simulink model "EV_BMS_SOC"  (R2024a)
settings: Solver=ode1  StartTime=0.0  StopTime=Tstop  FixedStep=Ts  RelTol=1e-3
InitFcn:
  | bms_simulink_init;
values from neighbouring files (symbols this model uses):
  I_max = P_.I_max    [bms_simulink_init.m]
  I_offset = P_.I_offset    [bms_simulink_init.m]
  inv_Cth = 1 / P_.Cth    [bms_simulink_init.m]
  inv_Rth = 1 / P_.Rth    [bms_simulink_init.m]
  k_soc = -100 / (3600 * Q_Ah)    [bms_simulink_init.m]
  OCV_pack = P.OCV_pack    [battery_voltage_model.m]    (also in bms_simulink_init.m = P_.OCV_pack)
  protection_enable = double(sc_.protection)    [bms_simulink_init.m]
  R0 = P_.R0    [bms_simulink_init.m]
  SOC_bp = P.SOC_bp    [battery_voltage_model.m]    (also in bms_simulink_init.m = P_.SOC_bp)
  SOC_init = sc_.SOC_init    [bms_simulink_init.m]
  T_init = sc_.T_init    [bms_simulink_init.m]
  T_max = P_.T_max    [bms_simulink_init.m]
  Ts = P_.dt    [bms_simulink_init.m]
  V_max = P_.V_max    [bms_simulink_init.m]
  V_min = P_.V_min    [bms_simulink_init.m]
undefined symbols (not defined in the file or in its folder): SOC_est_init, stage_select
settings Model: Creator=hp  LastModifiedBy=hp

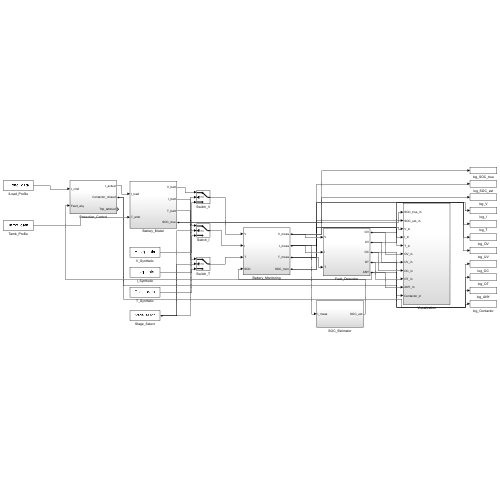
[thumbnail: Simulink's stored preview of the top-level diagram]
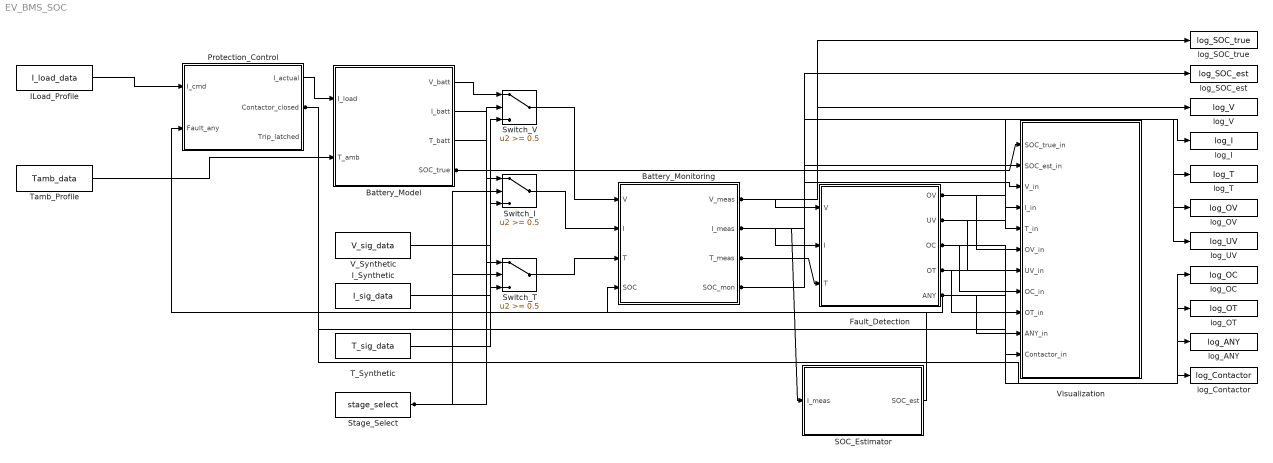
== system EV_BMS_SOC ==
  Battery_Model : Subsystem
  Battery_Monitoring : Subsystem
  Fault_Detection : Subsystem
  ILoad_Profile : FromWorkspace  VariableName=I_load_data  OutputAfterFinalValue=Holding final value
  I_Synthetic : FromWorkspace  VariableName=I_sig_data  OutputAfterFinalValue=Holding final value
  Protection_Control : Subsystem
  SOC_Estimator : Subsystem
  Stage_Select : Constant  Value=stage_select
  Switch_I : Switch  Threshold=0.5  SaturateOnIntegerOverflow=off  InputSameDT=off
  Switch_T : Switch  Threshold=0.5  SaturateOnIntegerOverflow=off  InputSameDT=off
  Switch_V : Switch  Threshold=0.5  SaturateOnIntegerOverflow=off  InputSameDT=off
  T_Synthetic : FromWorkspace  VariableName=T_sig_data  OutputAfterFinalValue=Holding final value
  Tamb_Profile : FromWorkspace  VariableName=Tamb_data  OutputAfterFinalValue=Holding final value
  V_Synthetic : FromWorkspace  VariableName=V_sig_data  OutputAfterFinalValue=Holding final value
  Visualization : Subsystem
  log_ANY : ToWorkspace  VariableName=log_ANY  SampleTime=-1
  log_Contactor : ToWorkspace  VariableName=log_Contactor  SampleTime=-1
  log_I : ToWorkspace  VariableName=log_I  SampleTime=-1
  log_OC : ToWorkspace  VariableName=log_OC  SampleTime=-1
  log_OT : ToWorkspace  VariableName=log_OT  SampleTime=-1
  log_OV : ToWorkspace  VariableName=log_OV  SampleTime=-1
  log_SOC_est : ToWorkspace  VariableName=log_SOC_est  SampleTime=-1
  log_SOC_true : ToWorkspace  VariableName=log_SOC_true  SampleTime=-1
  log_T : ToWorkspace  VariableName=log_T  SampleTime=-1
  log_UV : ToWorkspace  VariableName=log_UV  SampleTime=-1
  log_V : ToWorkspace  VariableName=log_V  SampleTime=-1
  wires:
  ILoad_Profile/1 -> Protection_Control/1(I_cmd)
  Protection_Control/1(I_actual) -> Battery_Model/1(I_load)
  Tamb_Profile/1 -> Battery_Model/2(T_amb)
  Battery_Model/1(V_batt) -> Switch_V/1
  V_Synthetic/1 -> Switch_V/3
  Stage_Select/1 -> Switch_V/2, Switch_I/2, Switch_T/2
  Battery_Model/2(I_batt) -> Switch_I/1
  I_Synthetic/1 -> Switch_I/3
  Battery_Model/3(T_batt) -> Switch_T/1
  T_Synthetic/1 -> Switch_T/3
  Switch_V/1 -> Battery_Monitoring/1(V)
  Switch_I/1 -> Battery_Monitoring/2(I)
  Switch_T/1 -> Battery_Monitoring/3(T)
  SOC_Estimator/1(SOC_est) -> Battery_Monitoring/4(SOC)
  Battery_Monitoring/2(I_meas) -> SOC_Estimator/1(I_meas), Fault_Detection/2(I), Visualization/4(I_in), log_I/1
  Battery_Monitoring/1(V_meas) -> Fault_Detection/1(V), Visualization/3(V_in), log_V/1
  Battery_Monitoring/3(T_meas) -> Fault_Detection/3(T), Visualization/5(T_in), log_T/1
  Fault_Detection/5(ANY) -> Protection_Control/2(Fault_any), Visualization/10(ANY_in), log_ANY/1
  Battery_Model/4(SOC_true) -> Visualization/1(SOC_true_in), log_SOC_true/1
  Battery_Monitoring/4(SOC_mon) -> Visualization/2(SOC_est_in), log_SOC_est/1
  Fault_Detection/1(OV) -> Visualization/6(OV_in), log_OV/1
  Fault_Detection/2(UV) -> Visualization/7(UV_in), log_UV/1
  Fault_Detection/3(OC) -> Visualization/8(OC_in), log_OC/1
  Fault_Detection/4(OT) -> Visualization/9(OT_in), log_OT/1
  Protection_Control/2(Contactor_closed) -> Visualization/11(Contactor_in), log_Contactor/1

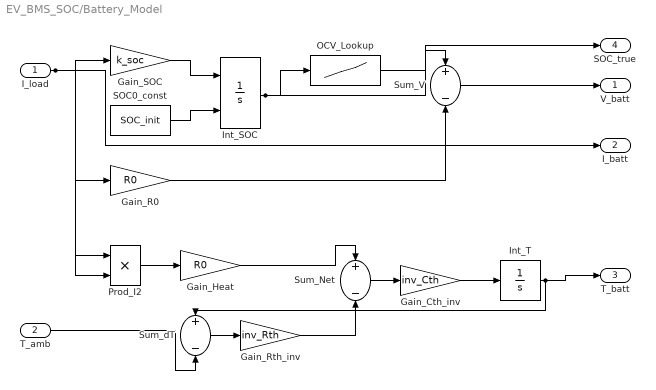
== system EV_BMS_SOC/Battery_Model ==
  I_load : Inport
  T_amb : Inport  Port=2
  Gain_Cth_inv : Gain  Gain=inv_Cth
  Gain_Heat : Gain  Gain=R0
  Gain_R0 : Gain  Gain=R0
  Gain_Rth_inv : Gain  Gain=inv_Rth
  Gain_SOC : Gain  Gain=k_soc
  Int_SOC : Integrator  InitialConditionSource=external  LimitOutput=on  UpperSaturationLimit=100  LowerSaturationLimit=0
  Int_T : Integrator  InitialCondition=T_init
  OCV_Lookup : Lookup_n-D  NumberOfTableDimensions=1  BreakpointsForDimension1=SOC_bp  Table=OCV_pack  ExtrapMethod=Clip  InternalRulePriority=Speed  RndMeth=Simplest
  Prod_I2 : Product
  SOC0_const : Constant  Value=SOC_init
  Sum_Net : Sum  Inputs=+-
  Sum_V : Sum  Inputs=+-
  Sum_dT : Sum  Inputs=+-
  V_batt : Outport
  I_batt : Outport  Port=2
  T_batt : Outport  Port=3
  SOC_true : Outport  Port=4
  wires:
  I_load/1 -> Gain_SOC/1, Gain_R0/1, I_batt/1, Prod_I2/1, Prod_I2/2
  Gain_SOC/1 -> Int_SOC/1
  SOC0_const/1 -> Int_SOC/2
  Int_SOC/1 -> OCV_Lookup/1, SOC_true/1
  OCV_Lookup/1 -> Sum_V/1
  Gain_R0/1 -> Sum_V/2
  Sum_V/1 -> V_batt/1
  Prod_I2/1 -> Gain_Heat/1
  Int_T/1 -> Sum_dT/1, T_batt/1
  T_amb/1 -> Sum_dT/2
  Sum_dT/1 -> Gain_Rth_inv/1
  Gain_Heat/1 -> Sum_Net/1
  Gain_Rth_inv/1 -> Sum_Net/2
  Sum_Net/1 -> Gain_Cth_inv/1
  Gain_Cth_inv/1 -> Int_T/1

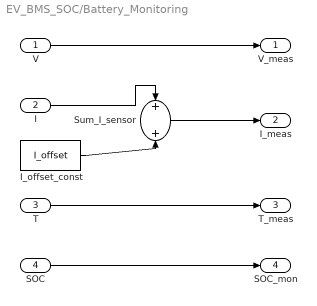
== system EV_BMS_SOC/Battery_Monitoring ==
  V : Inport
  I : Inport  Port=2
  T : Inport  Port=3
  SOC : Inport  Port=4
  I_offset_const : Constant  Value=I_offset
  Sum_I_sensor : Sum
  V_meas : Outport
  I_meas : Outport  Port=2
  T_meas : Outport  Port=3
  SOC_mon : Outport  Port=4
  wires:
  V/1 -> V_meas/1
  I/1 -> Sum_I_sensor/1
  I_offset_const/1 -> Sum_I_sensor/2
  Sum_I_sensor/1 -> I_meas/1
  T/1 -> T_meas/1
  SOC/1 -> SOC_mon/1

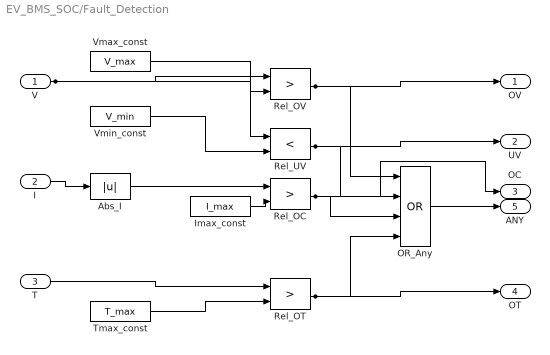
== system EV_BMS_SOC/Fault_Detection ==
  V : Inport
  I : Inport  Port=2
  T : Inport  Port=3
  Abs_I : Abs  SaturateOnIntegerOverflow=off
  Imax_const : Constant  Value=I_max
  OR_Any : Logic  Operator=OR  Inputs=4  AllPortsSameDT=off  OutDataTypeStr=boolean
  Rel_OC : RelationalOperator  Operator=>  OutDataTypeStr=boolean  RndMeth=Simplest  InputSameDT=off
  Rel_OT : RelationalOperator  Operator=>  OutDataTypeStr=boolean  RndMeth=Simplest  InputSameDT=off
  Rel_OV : RelationalOperator  Operator=>  OutDataTypeStr=boolean  RndMeth=Simplest  InputSameDT=off
  Rel_UV : RelationalOperator  Operator=<  OutDataTypeStr=boolean  RndMeth=Simplest  InputSameDT=off
  Tmax_const : Constant  Value=T_max
  Vmax_const : Constant  Value=V_max
  Vmin_const : Constant  Value=V_min
  OV : Outport
  UV : Outport  Port=2
  OC : Outport  Port=3
  OT : Outport  Port=4
  ANY : Outport  Port=5
  wires:
  V/1 -> Rel_OV/1, Rel_UV/1
  Vmax_const/1 -> Rel_OV/2
  Vmin_const/1 -> Rel_UV/2
  I/1 -> Abs_I/1
  Abs_I/1 -> Rel_OC/1
  Imax_const/1 -> Rel_OC/2
  T/1 -> Rel_OT/1
  Tmax_const/1 -> Rel_OT/2
  Rel_OV/1 -> OR_Any/1, OV/1
  Rel_UV/1 -> OR_Any/2, UV/1
  Rel_OC/1 -> OR_Any/3, OC/1
  Rel_OT/1 -> OR_Any/4, OT/1
  OR_Any/1 -> ANY/1

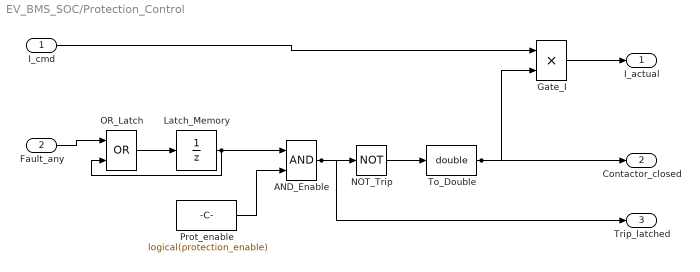
== system EV_BMS_SOC/Protection_Control ==
  I_cmd : Inport
  Fault_any : Inport  Port=2
  AND_Enable : Logic  AllPortsSameDT=off  OutDataTypeStr=boolean
  Gate_I : Product
  Latch_Memory : UnitDelay  SampleTime=Ts  HasFrameUpgradeWarning=on
  NOT_Trip : Logic  Operator=NOT  AllPortsSameDT=off  OutDataTypeStr=boolean
  OR_Latch : Logic  Operator=OR  AllPortsSameDT=off  OutDataTypeStr=boolean
  Prot_enable : Constant  Value=logical(protection_enable)  OutDataTypeStr=boolean
  To_Double : DataTypeConversion  OutDataTypeStr=double  SaturateOnIntegerOverflow=off  RndMeth=Floor
  I_actual : Outport
  Contactor_closed : Outport  Port=2
  Trip_latched : Outport  Port=3
  wires:
  Fault_any/1 -> OR_Latch/1
  OR_Latch/1 -> Latch_Memory/1
  Latch_Memory/1 -> OR_Latch/2, AND_Enable/1
  Prot_enable/1 -> AND_Enable/2
  AND_Enable/1 -> NOT_Trip/1, Trip_latched/1
  NOT_Trip/1 -> To_Double/1
  I_cmd/1 -> Gate_I/1
  To_Double/1 -> Gate_I/2, Contactor_closed/1
  Gate_I/1 -> I_actual/1

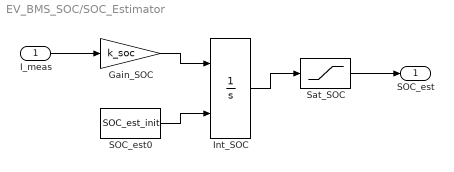
== system EV_BMS_SOC/SOC_Estimator ==
  I_meas : Inport
  Gain_SOC : Gain  Gain=k_soc
  Int_SOC : Integrator  InitialConditionSource=external  LimitOutput=on  UpperSaturationLimit=100  LowerSaturationLimit=0
  SOC_est0 : Constant  Value=SOC_est_init
  Sat_SOC : Saturate  UpperLimit=100  LowerLimit=0
  SOC_est : Outport
  wires:
  I_meas/1 -> Gain_SOC/1
  Gain_SOC/1 -> Int_SOC/1
  SOC_est0/1 -> Int_SOC/2
  Int_SOC/1 -> Sat_SOC/1
  Sat_SOC/1 -> SOC_est/1

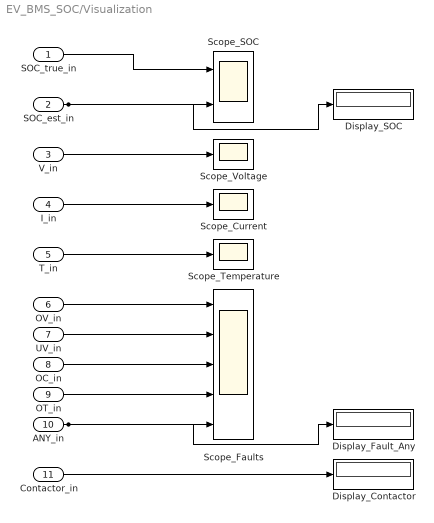
== system EV_BMS_SOC/Visualization ==
  SOC_true_in : Inport
  SOC_est_in : Inport  Port=2
  V_in : Inport  Port=3
  I_in : Inport  Port=4
  T_in : Inport  Port=5
  OV_in : Inport  Port=6
  UV_in : Inport  Port=7
  OC_in : Inport  Port=8
  OT_in : Inport  Port=9
  ANY_in : Inport  Port=10
  Contactor_in : Inport  Port=11
  Display_Contactor : Display
  Display_Fault_Any : Display
  Display_SOC : Display
  Scope_Current : Scope
  Scope_Faults : Scope  NumInputPorts=5
  Scope_SOC : Scope  NumInputPorts=2
  Scope_Temperature : Scope
  Scope_Voltage : Scope
  wires:
  SOC_true_in/1 -> Scope_SOC/1
  SOC_est_in/1 -> Scope_SOC/2, Display_SOC/1
  V_in/1 -> Scope_Voltage/1
  I_in/1 -> Scope_Current/1
  T_in/1 -> Scope_Temperature/1
  OV_in/1 -> Scope_Faults/1
  UV_in/1 -> Scope_Faults/2
  OC_in/1 -> Scope_Faults/3
  OT_in/1 -> Scope_Faults/4
  ANY_in/1 -> Scope_Faults/5, Display_Fault_Any/1
  Contactor_in/1 -> Display_Contactor/1
